simulink model "HarnessModel_CtrlEnv_Vehicle"  (R2026a)
settings: Solver=daessc  StopTime=300
PreLoadFcn:
  | HarnessSetup_CtrlEnv_Vehicle
libraries: simulink x1
settings Model: Creator=isaacito  LastModifiedBy=isaacito
settings SimscapeCC: SimscapeNominalValues="[{\"value\":\"1\",\"unit\":\"A\"},{\"value\":\"1\",\"unit\":\"bar\"},{\"value\":\"1\",\"unit\":\"cm^2\"},{\"value\":\"1\",\"unit\":\"cm^3/s\"},{\"value\":\"1\",\"unit\":\"kJ/kg\"},{\"value\":\"1\",\"unit\":\"kW\"},{\"value\":\"1\",\"unit\":\"l\"},{\"value\":\"1\",\"unit\":\"N\"},{\"value\":\"1\",\"unit\":\"N*m\"},{\"value\":\"1\",\"unit\":\"V\"}]"  SimscapeLogSimulationStatistics=on  SimscapeLogLimitData=off  SimscapeLogDataHistory=5000.0

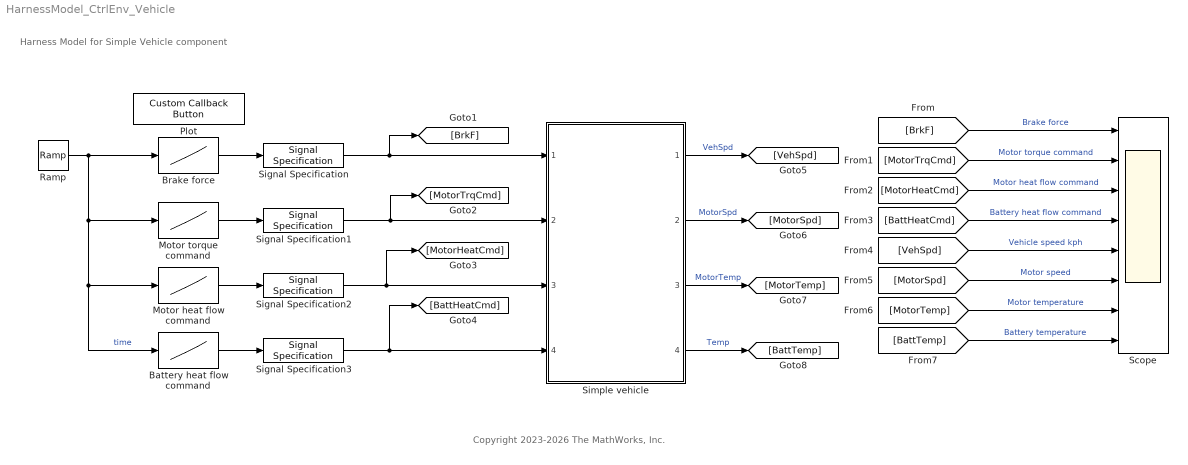
== system HarnessModel_CtrlEnv_Vehicle ==
  note: Copyright 2023-2026 The MathWorks, Inc.
  note: Harness Model for Simple Vehicle component
  Battery heat flow command : Lookup_n-D  NumberOfTableDimensions=1  BreakpointsForDimension1=[0; 45; 90; 110; 150; 190; 210; 255; 300]  Table=[0; 0; 0; -1000; -1000; -1000; 1000; 1000; 1000]  InterpMethod=Akima spline  InternalRulePriority=Speed  RndMeth=Simplest
  Brake force : Lookup_n-D  NumberOfTableDimensions=1  BreakpointsForDimension1=[0; 100; 200; 230; 255; 280]  Table=[0; 0; 0; 1000; 1000; 1000]  InterpMethod=Akima spline  InternalRulePriority=Speed  RndMeth=Simplest
  Motor heat flow command : Lookup_n-D  NumberOfTableDimensions=1  BreakpointsForDimension1=[0; 45; 90; 110; 150; 190; 210; 255; 300]  Table=[0; 0; 0; -1000; -1000; -1000; 1000; 1000; 1000]  InterpMethod=Akima spline  InternalRulePriority=Speed  RndMeth=Simplest
  Motor torque command : Lookup_n-D  NumberOfTableDimensions=1  BreakpointsForDimension1=[0; 50; 100; 110; 155; 200]  Table=[100; 100; 100; 0; 0; 0]  InterpMethod=Akima spline  InternalRulePriority=Speed  RndMeth=Simplest
  Plot : CustomCallbackButton  Configuration="{\"components\":[{\"name\":\"BackgroundImageComponent\",\"settings\":{\"image\":{\"size\":[0,0],\"src\":\"default\",\"srcOrientation\":\"Right\"},\"position\":[0,0,1,1]}},{\"name\":\"ButtonStateComponent\",\"settings\":{\"buttonType\":\"momentary\",\"clickFcn\":\"% Specify blocks to sort plot order.\\nblocks = [\\n  \\\"Brake force\\\"\\n  \\\"Motor torque command\\\"\\n  \\\"Motor heat flow command\\\"\\n  \\\"Battery heat flow command\\\"\\n];\\nbevutil1.SignalUtil.plotLookupTable1DBlocks(gcs, Blocks=blocks, DivisionType=\\\"InterpolationInterval\\\", InterpolationInterval=0.1)\",\"onValue\":1,\"position\":[0,0,1,1],\"pressDelay\":\"500\",\"pressFcn\":\"\",\"repeatInterval\":\"0\",\"states\":[{\"horizontalAlignment\":\"center\",\"image\":{\"position\":[0,0,1,1],\"size\":[1,1],\"src\":\"default\",\"srcOrientation\":\"Right\"},\"label\":{\"color\":[0.01176470588,0.01176470588,0.01176470588,1],\"icon\":{\"size\":[0,0],\"src\":\"default\",\"srcOrientation\":\"Right\"},\"iconOffset\":0,\"iconPlacement\":\"left\",\"opacity\":1,\"show\":true,\"text\":{\"content\":\"Lookup tables\",\"font\":\"Helvetica\"}},\"labelOffset\":[0,0],\"verticalAlignment\":\"middle\"},{\"horizontalAlignment\":\"center\",\"image\":{\"position\":[0,0,1,1],\"size\":[1,1],\"src\":\"default\",\"srcOrientation\":\"Right\"},\"label\":{\"color\":[0.01176470588,0.01176470588,0.01176470588,1],\"icon\":{\"size\":[0,0],\"src\":\"default\",\"srcOrientation\":\"Right\"},\"iconOffset\":0,\"iconPlacement\":\"left\",\"opacity\":1,\"show\":true,\"text\":{\"content\":\"Lookup tables\",\"font\":\"Helvetica\"}},\"labelOffset\":[0,0],\"verticalAlignment\":\"middle\"},{\"horizontalAlignment\":\"center\",\"image\":{\"position\":[0,0,1,1],\"size\":[1,1],\"src\":\"default\",\"srcOrientation\":\"Right\"},\"label\":{\"color\":[0.01176470588,0.01176470588,0.01176470588,1],\"icon\":{\"size\":[0,0],\"src\":\"default\",\"srcOrientation\":\"Right\"},\"iconOffset\":0,\"iconPlacement\":\"left\",\"opacity\":1,\"show\":true,\"text\":{\"content\":\"Lookup tables\",\"font\":\"Helvetica\"}},\"labelOffset\":[0,0],\"verticalAlignment\":\"middle\"},{\"horizontalAlignment\":\"center\",\"image\":{\"position\":[0,0,1,1],\"size\":[1,1],\"src\":\"default\",\"srcOrientation\":\"Right\"},\"label\":{\"color\":[0.01176470588,0.01176470588,0.01176470588,1],\"icon\":{\"size\":[0,0],\"src\":\"default\",\"srcOrientation\":\"Right\"},\"iconOffset\":0,\"iconPlacement\":\"left\",\"opacity\":1,\"show\":true,\"text\":{\"content\":\"Lookup tables\",\"font\":\"Helvetica\"}},\"labelOffset\":[0,0],\"verticalAlignment\":\"middle\"}]}},{\"name\":\"ForegroundImageComponent\",\"settings\":{\"image\":{\"size\":[0,0],\"src\":\"default\",\"srcOrientation\":\"Right\"},\"isForeground\":1,\"position\":[0,0,1,1]}}],\"derived\":{\"blockParameters\":{\"AutoActivate\":true,\"ButtonText\":\"Lookup tables\",\"ButtonType\":\"Momentary\",\"ClickFcn\":\"% Specify blocks to sort plot order.\\nblocks = [\\n  \\\"Brake force\\\"\\n  \\\"Motor torque command\\\"\\n  \\\"Motor heat flow command\\\"\\n  \\\"Battery heat flow command\\\"\\n];\\nbevutil1.SignalUtil.plotLookupTable1DBlocks(gcs, Blocks=blocks, DivisionType=\\\"InterpolationInterval\\\", InterpolationInterval=0.1)\",\"OnValue\":1,\"PressDelay\":\"500\",\"PressFcn\":\"\",\"RepeatInterval\":\"0\",\"fixedAspectRatio\":\"off\"}},\"settings\":{\"BindingType\":\"standalone\",\"autoActivate\":true,\"backgroundColor\":[244,244,244,1],\"backgroundOffset\":0.2,\"backgroundOpacity\":1,\"fixedAspectRatio\":\"off\",\"foregroundColor\":[0.01176470588,0.01176470588,0.01176470588,1],\"migratedFromLegacy\":true,\"useBackgroundColor\":true,\"variant\":\"callback\",\"version\":\"R2025a\"},\"type\":\"Button\"}"  CustomBackgroundColor="{\"color\":[0.9568627451,0.9568627451,0.9568627451],\"show\":true}"
  Ramp : simulink/Sources/Ramp  slope=1  start=0  InitialOutput=0
      settings: AttributesFormatString=|
      | Slope: %<slope>
      | Start time: %<start>
      | Initial output: %<InitialOutput>
  Scope : Scope  NumInputPorts=8
      settings: ActiveDisplayYMinimum=-124.99999999999997  ActiveDisplayYMaximum=1125
  Signal Specification : SignalSpecification  Unit=N
  Signal Specification1 : SignalSpecification  Unit=N*m
  Signal Specification2 : SignalSpecification  Unit=W
  Signal Specification3 : SignalSpecification  Unit=W
  Simple vehicle : Subsystem  ReferencedSubsystem=CtrlEnv_Vehicle_refsub
      settings: OpenFcn=|
      | % Look under mask:
      | open_system(gcb, "force")
  wires:
  Signal Specification/1 -> [BrkF], Simple vehicle/1
  Signal Specification1/1 -> [MotorTrqCmd], Simple vehicle/2
  Signal Specification2/1 -> [MotorHeatCmd], Simple vehicle/3
  Signal Specification3/1 -> [BattHeatCmd], Simple vehicle/4
  Simple vehicle/1 -> [VehSpd]  "VehSpd"
  Simple vehicle/2 -> [MotorSpd]  "MotorSpd"
  Simple vehicle/3 -> [MotorTemp]  "MotorTemp"
  Simple vehicle/4 -> [BattTemp]  "Temp"
  [BrkF] -> Scope/1  "Brake force"
  [MotorTrqCmd] -> Scope/2  "Motor torque command"
  [MotorHeatCmd] -> Scope/3  "Motor heat flow command"
  [BattHeatCmd] -> Scope/4  "Battery heat flow command"
  [VehSpd] -> Scope/5  "Vehicle speed kph"
  [MotorSpd] -> Scope/6  "Motor speed"
  [MotorTemp] -> Scope/7  "Motor temperature"
  [BattTemp] -> Scope/8  "Battery temperature"
  Brake force/1 -> Signal Specification/1
  Ramp/1 -> Motor heat flow command/1, Battery heat flow command/1, Motor torque command/1, Brake force/1  "time"
  Motor torque command/1 -> Signal Specification1/1
  Motor heat flow command/1 -> Signal Specification2/1
  Battery heat flow command/1 -> Signal Specification3/1
